simulink model "simulink_model"  (R2026b)
settings: Solver=VariableStepAuto  StopTime=30
values from neighbouring files (symbols this model uses):
  Vx_ini = 0    [Vehicle_Params.m]
undefined symbols (not defined in the file or in its folder): Fd_calculate_linear, Fx_calculate_linear, Fyf_calculate_linear, Fyr_calculate_linear, Vehicle_dynamics
settings Model: Creator=osganig  LastModifiedBy=osganig
settings RTWCC: GPUComputeCapability=5.0

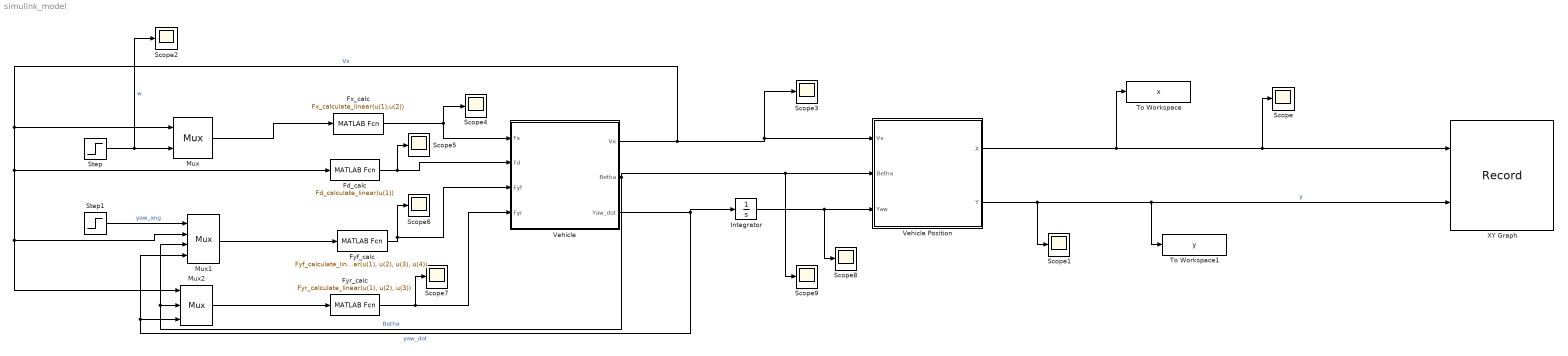
== system simulink_model ==
  Fd_calc : MATLABFcn  MATLABFcn=Fd_calculate_linear(u(1))  OutputDimensions=1
  Fx_calc : MATLABFcn  MATLABFcn=Fx_calculate_linear(u(1),u(2))
  Fyf_calc : MATLABFcn  MATLABFcn=Fyf_calculate_linear(u(1), u(2), u(3), u(4))
  Fyr_calc : MATLABFcn  MATLABFcn=Fyr_calculate_linear(u(1), u(2), u(3))
  Integrator : Integrator
  Mux : Mux  Inputs=2
      settings: DisplayOption=signals
  Mux1 : Mux
      settings: DisplayOption=signals
  Mux2 : Mux  Inputs=3
      settings: DisplayOption=signals
  Scope{,1..9} (10 alike) : Scope
      Scope settings: ActiveDisplayYMinimum=-25.572959735791361  ActiveDisplayYMaximum=31.952291021062504
      Scope1 settings: ActiveDisplayYMinimum=-5.9931566116679731  ActiveDisplayYMaximum=10.751762435245872
      Scope2 settings: ActiveDisplayYMinimum=-0.59720443572329618  ActiveDisplayYMaximum=7.9746237769541439  DataLoggingVariableName=ScopeData4
      Scope3 settings: ActiveDisplayYMinimum=-7.219792463547801  ActiveDisplayYMaximum=20.359698198515176  DataLoggingVariableName=ScopeData5
      Scope4 settings: ActiveDisplayYMinimum=-1659.1167868506818  ActiveDisplayYMaximum=86495.05147575686  DataLoggingVariableName=ScopeData6
      Scope5 settings: DataLoggingVariableName=ScopeData7
      Scope6 settings: ActiveDisplayYMinimum=-1.9098210806913427E+6  ActiveDisplayYMaximum=1.9746260675124722E+6  DataLoggingVariableName=ScopeData8
      Scope7 settings: ActiveDisplayYMinimum=-4.3524915288469438E+6  ActiveDisplayYMaximum=4.27967006501927E+6  DataLoggingVariableName=ScopeData9
      Scope8 settings: DataLoggingVariableName=ScopeData10
      Scope9 settings: DataLoggingVariableName=ScopeData11
  Step : Step  FinalValue=w_input  SampleTime=0
  Step1 : Step  Time=2  FinalValue=delta_input  SampleTime=0
  To Workspace : ToWorkspace  VariableName=x  SampleTime=-1
  To Workspace1 : ToWorkspace  VariableName=y  SampleTime=-1
  Vehicle : Subsystem
  Vehicle Position : Subsystem
  XY Graph : Record  NumPorts=2.0  FileSettingsInternal="{\"entries\":[{\"content\":{\"excelSettings\":{\"content\":{},\"type\":\"Streamout.ExcelSettings\"},\"parquetSettings\":{\"content\":{},\"type\":\"Streamout.ParquetSettings\"}},\"type\":\"Streamout.FileSettingStorage\",\"uuid\":\"\"}],\"packageUris\":[\"http:\\/\\/schema.mathworks.com\\/mf0\\/streamout_blocks\\/R2020a\"],\"version\":\"1.0\"}"  FrameSettings=[0, 0]  Layout=[1 1]  SignalsInternal="{\"entries\":[{\"content\":{\"signals\":[{\"content\":{\"blockPath\":[],\"dimensions\":[1],\"domain\":\"\",\"lineColor\":\"#a2142f\",\"plots\":[ 1 ],\"port\":1,\"sid\":[\"\"],\"signalID\":1,\"signalName\":\"Vehicle Position:1\"},\"type\":\"RecordBlkView.Signal\",\"uuid\":\"\"},{\"content\":{\"blockPath\":[],\"dimensions\":[1],\"domain\":\"\",\"lineColor\":\"#139fff\",\"plots\":[ 1 ],\"port\":2,\"sid\":[\"\"],\"signalID\":2,\"signalName\":\"y\"},\"type\":\"RecordBlkView.Signal\",\"uuid\":\"\"}]},\"type\":\"RecordBlkView.InputSignals\",\"uuid\":\"\"}],\"packageUris\":[\"http:\\/\\/schema.mathworks.com\\/mf0\\/streamout_blocks\\/R2020a\"],\"version\":\"1.0\"}"  VisualizationBindings="{\"xyplotplugin\":{\"info\":[{\"series\":[{\"bindingParametersList\":[{\"parameter\":\"X-Axis\",\"signalID\":1,\"signalName\":\"Vehicle Position:1\"},{\"parameter\":\"Y-Axis\",\"signalID\":2,\"signalName\":\"y\"}],\"seriesID\":0}],\"subplotID\":1}]}}"  CompatibilityTag=XY
  wires:
  Fyf_calc/1 -> Vehicle/3(Fyf), Scope6/1
  Fyr_calc/1 -> Scope7/1, Vehicle/4(Fyr)
  Fd_calc/1 -> Scope5/1, Vehicle/2(Fd)
  Vehicle/1(Vx) -> Mux2/1, Mux1/2, Fd_calc/1, Mux/1, Scope3/1, Vehicle Position/1(Vx)  "Vx"
  Vehicle/2(Betha) -> Scope9/1, Vehicle Position/2(Betha), Mux1/3, Mux2/2  "Betha"
  Vehicle/3(Yaw_dot) -> Integrator/1, Mux2/3, Mux1/4  "yaw_dot"
  Integrator/1 -> Scope8/1, Vehicle Position/3(Yaw)
  Vehicle Position/1(X) -> To Workspace/1, Scope/1, XY Graph/1
  Vehicle Position/2(Y) -> Scope1/1, To Workspace1/1, XY Graph/2  "y"
  Mux/1 -> Fx_calc/1
  Fx_calc/1 -> Scope4/1, Vehicle/1(Fx)
  Mux1/1 -> Fyf_calc/1
  Mux2/1 -> Fyr_calc/1
  Step/1 -> Scope2/1, Mux/2  "w"
  Step1/1 -> Mux1/1  "yaw_ang"

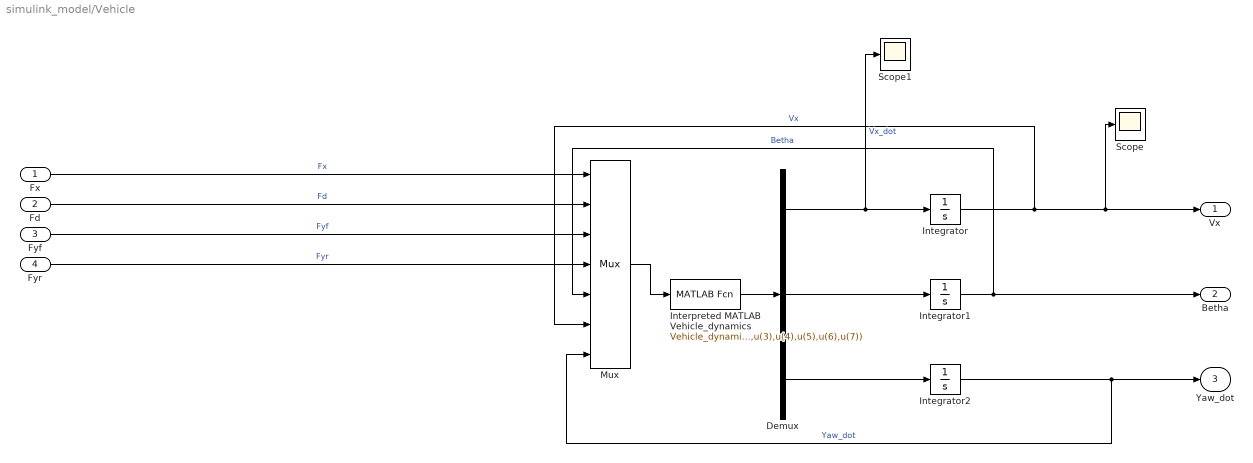
== system simulink_model/Vehicle ==
  Fx : Inport
  Fd : Inport  Port=2
  Fyf : Inport  Port=3
  Fyr : Inport  Port=4
  Demux : Demux  Outputs=3
  Integrator : Integrator  InitialCondition=Vx_ini
  Integrator1 : Integrator
  Integrator2 : Integrator
  Interpreted MATLAB Vehicle_dynamics : MATLABFcn  MATLABFcn=Vehicle_dynamics(u(1),u(2),u(3),u(4),u(5),u(6),u(7))  OutputDimensions=3
  Mux : Mux  Inputs=7
      settings: DisplayOption=signals
  Scope : Scope
      settings: ActiveDisplayYMinimum=-853712.461853775  ActiveDisplayYMaximum=812132.13991399459  DataLoggingVariableName=ScopeData2
  Scope1 : Scope
      settings: DataLoggingVariableName=ScopeData3
  Vx : Outport
  Betha : Outport  Port=2
  Yaw_dot : Outport  Port=3
  wires:
  Fx/1 -> Mux/1  "Fx"
  Fd/1 -> Mux/2  "Fd"
  Fyf/1 -> Mux/3  "Fyf"
  Fyr/1 -> Mux/4  "Fyr"
  Demux/1 -> Scope1/1, Integrator/1  "Vx_dot"
  Demux/2 -> Integrator1/1
  Demux/3 -> Integrator2/1
  Integrator2/1 -> Mux/7, Yaw_dot/1  "Yaw_dot"
  Integrator1/1 -> Mux/5, Betha/1  "Betha"
  Integrator/1 -> Mux/6, Scope/1, Vx/1  "Vx"
  Mux/1 -> Interpreted MATLAB Vehicle_dynamics/1
  Interpreted MATLAB Vehicle_dynamics/1 -> Demux/1

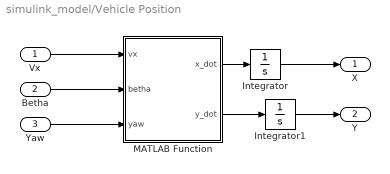
== system simulink_model/Vehicle Position ==
  Vx : Inport
  Betha : Inport  Port=2
  Yaw : Inport  Port=3
  Integrator : Integrator
  Integrator1 : Integrator
  MATLAB Function : MATLAB Function  TreatAsAtomicUnit=on
  X : Outport
  Y : Outport  Port=2
  wires:
  Vx/1 -> MATLAB Function/1(vx)
  Betha/1 -> MATLAB Function/2(betha)
  Yaw/1 -> MATLAB Function/3(yaw)
  MATLAB Function/1(x_dot) -> Integrator/1
  Integrator/1 -> X/1
  MATLAB Function/2(y_dot) -> Integrator1/1
  Integrator1/1 -> Y/1

== matlab function simulink_model/Vehicle Position/MATLAB Function ==
  data: vx input; betha input; x_dot output; yaw input; y_dot output
function [x_dot,y_dot] = fcn(vx,betha,yaw)

vy = vx* tan(betha);
x_dot = vx*cos(yaw) - vy*sin(yaw);
y_dot = vx*sin(yaw)  + vy*cos(yaw);
